simulink model "simulink_model_integrator"  (R2014b)
settings: Solver=ode45  SolverMode=SingleTasking  StartTime=0.0  StopTime=10.0  RelTol=1e-3
values from neighbouring files (symbols this model uses):
  x0 = [0; pi; 0; 0]    [extensive_example_ocp.m]    (also in minimal_example_closed_loop.m = x_sim(:,i); minimal_example_ocp.m; minimal_example_sim.m = [0; 1e-1; 0; 0])
settings Model: CovMetricSettings=dwe  CovHtmlReporting=off  covSaveCumulativeToWorkspaceVar=off  CovSaveSingleToWorkspaceVar=off  CovExternalEMLEnable=on  CovSFcnEnable=on  Creator=oj  LastModifiedBy=PBM
settings DataIOCC: LimitDataPoints=off  SaveFormat=StructureWithTime  ReturnWorkspaceOutputs=on
settings DebuggingCC: SolverPrmCheckMsg=none  FrameProcessingCompatibilityMsg=error  SFUnexpectedBacktrackingDiag=error  SFNoUnconditionalDefaultTransitionDiag=error
settings HardwareCC: ProdBitPerPointer=64  ProdLargestAtomicFloat=Float  ProdIntDivRoundTo=Zero  ProdEndianess=LittleEndian  ProdHWDeviceType=Specified
settings ModelReferenceCC: PropagateSignalLabelsOutOfModel=on
settings SFSimCC: SimUseLocalCustomCode=on
settings RTWCC: RTWUseLocalCustomCode=on
settings GRTTargetCC: TargetLangStandard=C99 (ISO)

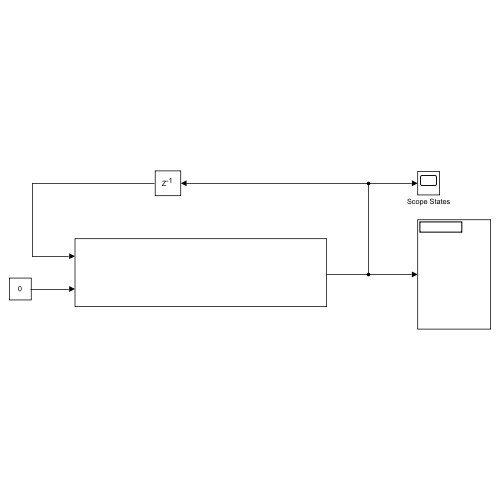
[thumbnail: Simulink's stored preview of the top-level diagram]
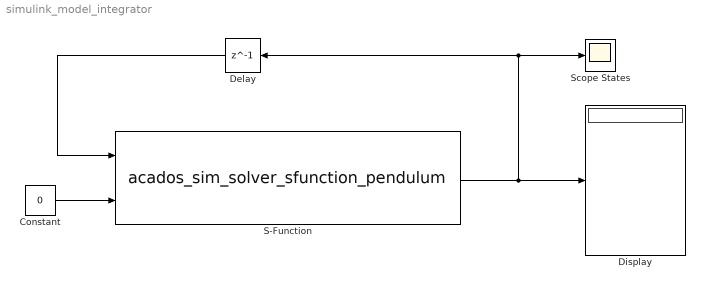
== system simulink_model_integrator ==
  Constant : Constant  Value=0
  Delay : Delay  DelayLength=1  InitialCondition=x0 + [0, 1, 0, 0]'  SampleTime=1/20
  Display : Display
  S-Function : S-Function  FunctionName=acados_sim_solver_sfunction_pendulum  SFunctionDeploymentMode=off  EnableBusSupport=off
      mask Display:
      | global sfun_sim_input_names sfun_sim_output_names
      | for i = 1:length(sfun_sim_input_names)
      | 	port_label('input', i, sfun_sim_input_names{i})
      | end
      | for i = 1:length(sfun_sim_output_names)
      | 	port_label('output', i, sfun_sim_output_names{i})
      | end
  Scope States : Scope
      settings: TimeRange=auto  MaxDataPoints=5000  SaveToWorkspace=off  SaveName=ScopeData  YMin=-4.47908  YMax=5.09937  SampleTime=-1
  wires:
  Constant/1 -> S-Function/2
  Delay/1 -> S-Function/1
  S-Function/1 -> Scope States/1, Delay/1, Display/1
